simulink model "MMC_1ph_Grid_ArmLeaders_EnergyBalancing_v3_1A"  (R2024a)
settings: Solver=FixedStepDiscrete  StartTime=0.0  StopTime=1  FixedStep=Ts  RelTol=1e-3
PreLoadFcn:
  | VDC=800; N=8; C=2.2e-3; vo=100; W_nom=0.5*C*N*vo^2;
  | Larm=5e-3; Rarm=0.5; f=50;
  | Vg_rms=230; Vg_pk=Vg_rms*sqrt(2); Lg=2e-3; Rg=0.1;
  | Pstar=1500; Qstar=0;
  | fsw=1250; Ts=1e-5; Ts_ctrl=1e-4; Cf=10e-6; Rf=10;
InitFcn:
  | VDC=800; N=8; C=2.2e-3; vo=100; W_nom=0.5*C*N*vo^2;
  | Larm=5e-3; Rarm=0.5; f=50;
  | Vg_rms=230; Vg_pk=Vg_rms*sqrt(2); Lg=2e-3; Rg=0.1;
  | Pstar=1500; Qstar=0;
  | fsw=1250; Ts=1e-5; Ts_ctrl=1e-4; Cf=10e-6; Rf=10;
libraries: spsHalfBridgeMMCLib x16, spsSeriesRLCBranchLib x4, spsCurrentMeasurementLib x3, spsGroundLib x2, spsDCVoltageSourceLib x2, spsACVoltageSourceLib x1, spspowerguiLib x1, spsVoltageMeasurementLib x1
(part 2 of 2)

== matlab function MMC_1ph_Grid_ArmLeaders_EnergyBalancing_v3_1A/SM_l7/Local Ctrl ==
  data: sm_id input; S_top output; m_arm input; i_arm input; Vc_i input; Vc_prev input; Vc_next input; t input; S_bot output
function [S_top, S_bot] = hb_sm_local_ctrl(sm_id, m_arm, i_arm, Vc_i, Vc_prev, Vc_next, t)
%#codegen
% ============ SUBMODULE LAYER : local voltage balancing + PSC-PWM ============
% Fully local: own capacitor voltage, the two ring neighbours, the arm modulation
% index, the arm current (sign only) and the time base.  No sorting and no access
% to the full Vc vector.  Executes at Ts (10 us).

N      = 8;         % SMs per arm  -> carrier phase shift (sm_id-1)/N
fsw    = 1250;      % carrier frequency per SM -> N*fsw = 10 kHz effective per arm
k_v    = 0.2;       % balancing gain (1/V)
dead   = 0.1;       % V, dead-band against chattering
Iscale = 1.0;       % A, smooth sign of the arm current

%% 1. neighbour-average consensus correction
err  = 0.5*(Vc_prev + Vc_next) - Vc_i;
if abs(err) < dead, err = 0; end
dirn = tanh(i_arm/Iscale);    % > 0 : inserting charges C  (both arms: i measured top -> bottom)
dm   = k_v*err*dirn;
m_i  = min(max(m_arm + dm, 0), 1);

%% 2. phase-shifted triangular carrier (0 -> 1 -> 0)
tau = mod(t*fsw + (sm_id - 1)/N, 1);
car = 1 - abs(2*tau - 1);

%% 3. half-bridge gating
if m_i >= car
    S_top = 1; S_bot = 0;     % insert  (+Vc)
else
    S_top = 0; S_bot = 1;     % bypass  (0 V)
end
end

== matlab function MMC_1ph_Grid_ArmLeaders_EnergyBalancing_v3_1A/SM_u8/Neighbors ==
  data: Vc_arm input; Vc_i output; i input; Vc_prev output; Vc_next output
function [Vc_i, Vc_prev, Vc_next] = get_neighbors(Vc_arm, i)
%#codegen
% Models the neighbour-to-neighbour link of the ring: returns the own capacitor
% voltage and the voltages of the previous / next (circular) neighbours.
% Only these three scalars reach the local controller.
N = length(Vc_arm);
k = min(max(round(i), 1), N);
Vc_i = Vc_arm(k);
if k == 1
    Vc_prev = Vc_arm(N);      % circular: SM1's previous neighbour is SMN
    Vc_next = Vc_arm(2);
elseif k == N
    Vc_prev = Vc_arm(N-1);
    Vc_next = Vc_arm(1);      % circular: SMN's next neighbour is SM1
else
    Vc_prev = Vc_arm(k-1);
    Vc_next = Vc_arm(k+1);
end
end

== matlab function MMC_1ph_Grid_ArmLeaders_EnergyBalancing_v3_1A/SM_u8/Local Ctrl ==
  data: sm_id input; S_top output; m_arm input; i_arm input; Vc_i input; Vc_prev input; Vc_next input; t input; S_bot output
function [S_top, S_bot] = hb_sm_local_ctrl(sm_id, m_arm, i_arm, Vc_i, Vc_prev, Vc_next, t)
%#codegen
% ============ SUBMODULE LAYER : local voltage balancing + PSC-PWM ============
% Fully local: own capacitor voltage, the two ring neighbours, the arm modulation
% index, the arm current (sign only) and the time base.  No sorting and no access
% to the full Vc vector.  Executes at Ts (10 us).

N      = 8;         % SMs per arm  -> carrier phase shift (sm_id-1)/N
fsw    = 1250;      % carrier frequency per SM -> N*fsw = 10 kHz effective per arm
k_v    = 0.2;       % balancing gain (1/V)
dead   = 0.1;       % V, dead-band against chattering
Iscale = 1.0;       % A, smooth sign of the arm current

%% 1. neighbour-average consensus correction
err  = 0.5*(Vc_prev + Vc_next) - Vc_i;
if abs(err) < dead, err = 0; end
dirn = tanh(i_arm/Iscale);    % > 0 : inserting charges C  (both arms: i measured top -> bottom)
dm   = k_v*err*dirn;
m_i  = min(max(m_arm + dm, 0), 1);

%% 2. phase-shifted triangular carrier (0 -> 1 -> 0)
tau = mod(t*fsw + (sm_id - 1)/N, 1);
car = 1 - abs(2*tau - 1);

%% 3. half-bridge gating
if m_i >= car
    S_top = 1; S_bot = 0;     % insert  (+Vc)
else
    S_top = 0; S_bot = 1;     % bypass  (0 V)
end
end

== matlab function MMC_1ph_Grid_ArmLeaders_EnergyBalancing_v3_1A/SM_l8/Neighbors ==
  data: Vc_arm input; Vc_i output; i input; Vc_prev output; Vc_next output
function [Vc_i, Vc_prev, Vc_next] = get_neighbors(Vc_arm, i)
%#codegen
% Models the neighbour-to-neighbour link of the ring: returns the own capacitor
% voltage and the voltages of the previous / next (circular) neighbours.
% Only these three scalars reach the local controller.
N = length(Vc_arm);
k = min(max(round(i), 1), N);
Vc_i = Vc_arm(k);
if k == 1
    Vc_prev = Vc_arm(N);      % circular: SM1's previous neighbour is SMN
    Vc_next = Vc_arm(2);
elseif k == N
    Vc_prev = Vc_arm(N-1);
    Vc_next = Vc_arm(1);      % circular: SMN's next neighbour is SM1
else
    Vc_prev = Vc_arm(k-1);
    Vc_next = Vc_arm(k+1);
end
end

== matlab function MMC_1ph_Grid_ArmLeaders_EnergyBalancing_v3_1A/SM_l8/Local Ctrl ==
  data: sm_id input; S_top output; m_arm input; i_arm input; Vc_i input; Vc_prev input; Vc_next input; t input; S_bot output
function [S_top, S_bot] = hb_sm_local_ctrl(sm_id, m_arm, i_arm, Vc_i, Vc_prev, Vc_next, t)
%#codegen
% ============ SUBMODULE LAYER : local voltage balancing + PSC-PWM ============
% Fully local: own capacitor voltage, the two ring neighbours, the arm modulation
% index, the arm current (sign only) and the time base.  No sorting and no access
% to the full Vc vector.  Executes at Ts (10 us).

N      = 8;         % SMs per arm  -> carrier phase shift (sm_id-1)/N
fsw    = 1250;      % carrier frequency per SM -> N*fsw = 10 kHz effective per arm
k_v    = 0.2;       % balancing gain (1/V)
dead   = 0.1;       % V, dead-band against chattering
Iscale = 1.0;       % A, smooth sign of the arm current

%% 1. neighbour-average consensus correction
err  = 0.5*(Vc_prev + Vc_next) - Vc_i;
if abs(err) < dead, err = 0; end
dirn = tanh(i_arm/Iscale);    % > 0 : inserting charges C  (both arms: i measured top -> bottom)
dm   = k_v*err*dirn;
m_i  = min(max(m_arm + dm, 0), 1);

%% 2. phase-shifted triangular carrier (0 -> 1 -> 0)
tau = mod(t*fsw + (sm_id - 1)/N, 1);
car = 1 - abs(2*tau - 1);

%% 3. half-bridge gating
if m_i >= car
    S_top = 1; S_bot = 0;     % insert  (+Vc)
else
    S_top = 0; S_bot = 1;     % bypass  (0 V)
end
end

== matlab function MMC_1ph_Grid_ArmLeaders_EnergyBalancing_v3_1A/Meas Filter MA10 ==
  data: v_ac input; v_ac_f output; i_ac input; i_u input; i_l input; i_ac_f output; i_u_f output; i_l_f output
function [v_ac_f, i_ac_f, i_u_f, i_l_f] = meas_avg(v_ac, i_ac, i_u, i_l)
%#codegen
% Measurement conditioning for the 10 kHz control layer.
% 10-sample boxcar at Ts = 10 us  ->  exact nulls at 10 kHz (= N*fsw, the dominant
% PWM ripple of each arm) and at its multiples, so the Rate Transition blocks that
% follow do not alias the switching ripple into the control loops.
M = 10;
persistent buf idx
if isempty(buf), buf = zeros(M,4); idx = 1; end
buf(idx,:) = [v_ac, i_ac, i_u, i_l];
idx = idx + 1; if idx > M, idx = 1; end
y = sum(buf,1)/M;
v_ac_f = y(1);
i_ac_f = y(2);
i_u_f  = y(3);
i_l_f  = y(4);
end

== matlab function MMC_1ph_Grid_ArmLeaders_EnergyBalancing_v3_1A/Arm Leader UPPER/Outer Loop ==
  data: v_ac input; i_ac_ref output; i_ac input; Pstar input; Qstar input; t input; theta output; V_amp output; P_meas output; Q_meas output
function [i_ac_ref, theta, V_amp, P_meas, Q_meas] = mmc_outer_ctrl(v_ac, i_ac, Pstar, Qstar, t)
%#codegen
% ================= OUTER LOOP - GRID-CONNECTED P/Q CONTROL (one instance per arm) =================
% Executes at Ts_ctrl (Rate Transition blocks on every input pin the rate).
% Both arm leaders run this same deterministic code on the same measurements, so
% they produce an identical i_ac_ref without exchanging anything.
%
%   SOGI on v_ac and i_ac -> orthogonal (alpha, beta) components
%   SOGI-PLL (normalised)  -> theta locked to the PCC voltage (v_alpha = V_amp*cos(theta))
%   P = 0.5*(va*ia + vb*ib) ,  Q = 0.5*(va*ib - vb*ia)   [Q > 0 : current LEADS voltage, capacitive]
%   i_ac_ref = Ip*cos(theta) - Iq*sin(theta)
%
%   USE_PLL = false falls back to an internal 50 Hz oscillator (standalone resistive load).

Ts      = 1e-4;              % execution period (s) == Ts_ctrl in the workspace
f0      = 50;  w0 = 2*pi*f0;
USE_PLL = true;              % true : grid-connected (PLL on v_ac)   false : internal oscillator
NMA     = 200;               % 20 ms moving average on P and Q (nulls 50/100 Hz residuals)
T_START = 0.15;              % s, references held at zero until the PLL has locked
PQ_RAMP = 10000;             % W/s (var/s), reference ramp after T_START (soft start)

% --- SOGI and PLL
k_sogi  = 1.41;              % SOGI gain -> bandwidth ~ k*f0/2 = 35 Hz
Kp_pll  = 50;  Ki_pll = 1000;   % on vq/V_amp (p.u.) -> wn = 32 rad/s (5 Hz), zeta = 0.79
dw_max  = 2*pi*5;            % rad/s, PLL integrator limit (+-5 Hz)

% --- P and Q loops (plant: P = 0.5*V_amp*Ip, ~163 W/A at 325 V) -> f_bw ~ 5 Hz
Kp_pq   = 0.004;             % A/W   (loop gain 0.65 with the 10 ms MA delay)
Ki_pq   = 0.2;               % A/(W*s)
I_max   = 15;                % A, amplitude limit of each current component
P_max   = 3000;              % W
Q_max   = 2000;              % var
tau_v   = 0.01;              % s, LPF on the SOGI magnitude

persistent th pll_i vs1 vs2 is1 is2 Vf bufP bufQ idx xi_p xi_q
if isempty(th)
    th = 0; pll_i = 0; vs1 = 0; vs2 = 0; is1 = 0; is2 = 0; Vf = 300;
    bufP = zeros(NMA,1); bufQ = zeros(NMA,1); idx = 1;
    xi_p = 0; xi_q = 0;
end

%% 1. SOGI (voltage and current), symplectic Euler at 10 kHz (unity gain at w0; forward Euler gives +2.3 %)
vs1 = vs1 + Ts*(k_sogi*w0*(v_ac - vs1) - w0*vs2);
vs2 = vs2 + Ts*w0*vs1;
is1 = is1 + Ts*(k_sogi*w0*(i_ac - is1) - w0*is2);
is2 = is2 + Ts*w0*is1;
va = vs1; vb = vs2; ia = is1; ib = is2;

%% 2. amplitude and angle
Vn = max(sqrt(va^2 + vb^2), 20);
Vf = Vf + (Ts/(tau_v + Ts))*(Vn - Vf);
V_amp = Vf;
if USE_PLL
    vq    = (-sin(th)*va + cos(th)*vb)/Vn;            % normalised q-axis error (p.u.)
    pll_i = min(max(pll_i + Ki_pll*Ts*vq, -dw_max), dw_max);
    th    = mod(th + (w0 + Kp_pll*vq + pll_i)*Ts, 2*pi);
else
    th    = mod(w0*t, 2*pi);
end
theta = th;

%% 3. measured P and Q (instantaneous from alpha/beta, then 20 ms average)
bufP(idx) = 0.5*(va*ia + vb*ib);
bufQ(idx) = 0.5*(va*ib - vb*ia);
idx = idx + 1; if idx > NMA, idx = 1; end
P_meas = sum(bufP)/NMA;
Q_meas = sum(bufQ)/NMA;

%% 4. P and Q loops -> current components (feed-forward + PI, clamping anti-windup)
if t < T_START
    P_use = 0; Q_use = 0;                             % wait for PLL lock
else
    lim   = PQ_RAMP*(t - T_START);                    % ramped envelope
    P_use = min(max(min(max(Pstar, -P_max), P_max), -lim), lim);
    Q_use = min(max(min(max(Qstar, -Q_max), Q_max), -lim), lim);
end
Ip_ff = 2*P_use/V_amp;   Iq_ff = 2*Q_use/V_amp;
e_p = P_use - P_meas;    e_q = Q_use - Q_meas;
Ip_un = Ip_ff + Kp_pq*e_p + xi_p;
if abs(Ip_un) < I_max, xi_p = min(max(xi_p + Ki_pq*Ts*e_p, -I_max), I_max); end
Iq_un = Iq_ff + Kp_pq*e_q + xi_q;
if abs(Iq_un) < I_max, xi_q = min(max(xi_q + Ki_pq*Ts*e_q, -I_max), I_max); end
Ip = min(max(Ip_un, -I_max), I_max);
Iq = min(max(Iq_un, -I_max), I_max);

%% 5. AC current reference
i_ac_ref = Ip*cos(theta) - Iq*sin(theta);
end

== matlab function MMC_1ph_Grid_ArmLeaders_EnergyBalancing_v3_1A/SM_l1/Neighbors ==
  data: Vc_arm input; Vc_i output; i input; Vc_prev output; Vc_next output
function [Vc_i, Vc_prev, Vc_next] = get_neighbors(Vc_arm, i)
%#codegen
% Models the neighbour-to-neighbour link of the ring: returns the own capacitor
% voltage and the voltages of the previous / next (circular) neighbours.
% Only these three scalars reach the local controller.
N = length(Vc_arm);
k = min(max(round(i), 1), N);
Vc_i = Vc_arm(k);
if k == 1
    Vc_prev = Vc_arm(N);      % circular: SM1's previous neighbour is SMN
    Vc_next = Vc_arm(2);
elseif k == N
    Vc_prev = Vc_arm(N-1);
    Vc_next = Vc_arm(1);      % circular: SMN's next neighbour is SM1
else
    Vc_prev = Vc_arm(k-1);
    Vc_next = Vc_arm(k+1);
end
end

== matlab function MMC_1ph_Grid_ArmLeaders_EnergyBalancing_v3_1A/Arm Leader UPPER/Inner Loop and Energy Balancing ==
  data: i_ac_ref input; m_arm output; theta input; V_amp input; P_meas input; v_ac input; i_arm input; Vc_arm input; W_other input; IsUpper input; Vdc input; Vc_nom input; W_arm output; dbg output
function [m_arm, W_arm, dbg] = mmc_arm_ctrl(i_ac_ref, theta, V_amp, P_meas, v_ac, i_arm, Vc_arm, W_other, IsUpper, Vdc, Vc_nom)
%#codegen
% ========== INNER LOOP + INTER-ARM ENERGY BALANCING  (one instance per arm) ==========
% Executes at Ts_ctrl.  The only information this arm needs from the OTHER arm is
% one scalar: its raw stored energy W_other (received through a one-period unit
% delay that models the communication latency).  With s = +1 (upper) / -1 (lower)
% both leaders compute the SAME i_circ_ref, so no further coordination is needed.
%
%   m_arm : modulation index of this arm (0..1)      -> SM layer (local PSC-PWM)
%   W_arm : raw energy of this arm (J)               -> sent to the other arm
%   dbg   : [i_ref; i_circ_ref; v_arm_ref; W_own_f; W_other_f]
%   Vdc, Vc_nom : DC-link voltage and nominal SM voltage, read from the workspace (VDC, vo)
%                 through Constant blocks.  N*Vc_nom may exceed Vdc (stack margin for |v_ac| -> Vdc/2).

Ts     = 1e-4;
C      = 2.2e-3;
N      = numel(Vc_arm);
w0     = 2*pi*50;
NMA    = 200;                 % 20 ms moving average on the energies (nulls 50/100 Hz)

% --- arm current loop: PI + resonant terms at 50 Hz and 100 Hz (plant L = 5 mH, R = 0.5 ohm) -> f_bw ~ 380 Hz
Kp_i = 12;    Ki_i = 1200;    Kr_i = 300;   xi_i_max = 300;   xr_max = 200;   v_pi_max = 400;
% --- CCSC: resonant term at 2*w0 removes the 100 Hz circulating current from THIS arm's current.
%     i_ref carries no 2w0 component, so any 2w0 content of i_arm is error -> driven to zero locally,
%     without knowing the other arm's current (single-phase equivalent of the dq -2w CCSC).
USE_CCSC = true;   Kr_2 = 300;   xr2_max = 150;
% --- total-energy loop  (dW_sum/dt = Vdc*i_dc - P_ac)          -> f_bw ~ 4 Hz
Kp_s = 0.03;  Ki_s = 0.3;     xi_s_max = 3;     i_dc_max  = 5;
% --- differential-energy loop (dW_dif/dt = -V_amp*I_dif)       -> wn ~ 12 rad/s, critically damped
Kp_d = 25;    Ki_d = 150;     xi_d_max = 300;   I_dif_max = 3;

persistent xi_i xr1 xr2 xc1 xc2 xi_s xi_d bufO bufX idx
if isempty(xi_i)
    xi_i = 0; xr1 = 0; xr2 = 0; xc1 = 0; xc2 = 0; xi_s = 0; xi_d = 0;
    W0   = 0.5*C*N*Vc_nom^2;
    bufO = W0*ones(NMA,1); bufX = W0*ones(NMA,1); idx = 1;
end
if IsUpper > 0.5, s = 1; else, s = -1; end

%% 1. own arm energy (raw) -> exported to the other arm
W_arm = 0.5*C*sum(Vc_arm.^2);
W_nom = 0.5*C*N*Vc_nom^2;

%% 2. energy filtering (both arms use identical filters -> identical results)
bufO(idx) = W_arm;
bufX(idx) = W_other;
idx = idx + 1; if idx > NMA, idx = 1; end
Wo = sum(bufO)/NMA;           % own   (filtered)
Wx = sum(bufX)/NMA;           % other (filtered)

%% 3. energy-balancing layer
% 3a. total energy -> DC circulating current (identical in both arms)
e_sum   = 2*W_nom - (Wo + Wx);
i_dc_un = P_meas/Vdc + Kp_s*e_sum + xi_s;                        % unsaturated
if abs(i_dc_un) < i_dc_max                                       % clamping anti-windup
    xi_s = min(max(xi_s + Ki_s*Ts*e_sum, -xi_s_max), xi_s_max);
end
i_dc_ref = min(max(i_dc_un, -i_dc_max), i_dc_max);

% 3b. differential energy (own - other) -> fundamental circulating current in phase
%     with v_ac.  s flips the sign so that both arms demand the SAME I_dif:
%     upper: +K*(Wu-Wl)   lower: -K*(Wl-Wu) = +K*(Wu-Wl)
e_dif    = Wo - Wx;
u_dif    = Kp_d*e_dif + xi_d;                                    % W
I_dif_un = s*u_dif/max(V_amp, 50);                               % A (unsaturated)
if abs(I_dif_un) < I_dif_max                                     % clamping anti-windup
    xi_d = min(max(xi_d + Ki_d*Ts*e_dif, -xi_d_max), xi_d_max);
end
I_dif = min(max(I_dif_un, -I_dif_max), I_dif_max);
i_circ_ref = i_dc_ref + I_dif*cos(theta);

%% 4. arm current reference and inner PI + R
%     i_u = +i_ac/2 + i_circ ,  i_l = -i_ac/2 + i_circ   (both measured top -> bottom)
i_ref = s*0.5*i_ac_ref + i_circ_ref;
err_i = i_ref - i_arm;
xi_i  = min(max(xi_i + Ki_i*Ts*err_i, -xi_i_max), xi_i_max);
% resonant integrator at w0 (symplectic Euler: |lambda| = 1, no drift)
xr1   = xr1 + Ts*(Kr_i*err_i - w0*xr2);
xr2   = xr2 + Ts*w0*xr1;
xr1   = min(max(xr1, -xr_max), xr_max);
% resonant integrator at 2*w0 (CCSC)
if USE_CCSC
    xc1 = xc1 + Ts*(Kr_2*err_i - 2*w0*xc2);
    xc2 = xc2 + Ts*2*w0*xc1;
    xc1 = min(max(xc1, -xr2_max), xr2_max);
else
    xc1 = 0; xc2 = 0;
end
v_pi  = min(max(Kp_i*err_i + xi_i + xr1 + xc1, -v_pi_max), v_pi_max);

%% 5. arm voltage reference -> modulation index
%     upper: v_u = Vdc/2 - v_ac - v_pi      lower: v_l = Vdc/2 + v_ac - v_pi
v_arm_ref = Vdc/2 - s*v_ac - v_pi;
V_stack   = max(sum(Vc_arm), 0.5*N*Vc_nom);        % measured stack voltage
m_arm     = min(max(v_arm_ref/V_stack, 0), 1);

dbg = [i_ref; i_circ_ref; v_arm_ref; Wo; Wx];
end

== matlab function MMC_1ph_Grid_ArmLeaders_EnergyBalancing_v3_1A/Arm Leader LOWER/Outer Loop ==
  data: v_ac input; i_ac_ref output; i_ac input; Pstar input; Qstar input; t input; theta output; V_amp output; P_meas output; Q_meas output
function [i_ac_ref, theta, V_amp, P_meas, Q_meas] = mmc_outer_ctrl(v_ac, i_ac, Pstar, Qstar, t)
%#codegen
% ================= OUTER LOOP - GRID-CONNECTED P/Q CONTROL (one instance per arm) =================
% Executes at Ts_ctrl (Rate Transition blocks on every input pin the rate).
% Both arm leaders run this same deterministic code on the same measurements, so
% they produce an identical i_ac_ref without exchanging anything.
%
%   SOGI on v_ac and i_ac -> orthogonal (alpha, beta) components
%   SOGI-PLL (normalised)  -> theta locked to the PCC voltage (v_alpha = V_amp*cos(theta))
%   P = 0.5*(va*ia + vb*ib) ,  Q = 0.5*(va*ib - vb*ia)   [Q > 0 : current LEADS voltage, capacitive]
%   i_ac_ref = Ip*cos(theta) - Iq*sin(theta)
%
%   USE_PLL = false falls back to an internal 50 Hz oscillator (standalone resistive load).

Ts      = 1e-4;              % execution period (s) == Ts_ctrl in the workspace
f0      = 50;  w0 = 2*pi*f0;
USE_PLL = true;              % true : grid-connected (PLL on v_ac)   false : internal oscillator
NMA     = 200;               % 20 ms moving average on P and Q (nulls 50/100 Hz residuals)
T_START = 0.15;              % s, references held at zero until the PLL has locked
PQ_RAMP = 10000;             % W/s (var/s), reference ramp after T_START (soft start)

% --- SOGI and PLL
k_sogi  = 1.41;              % SOGI gain -> bandwidth ~ k*f0/2 = 35 Hz
Kp_pll  = 50;  Ki_pll = 1000;   % on vq/V_amp (p.u.) -> wn = 32 rad/s (5 Hz), zeta = 0.79
dw_max  = 2*pi*5;            % rad/s, PLL integrator limit (+-5 Hz)

% --- P and Q loops (plant: P = 0.5*V_amp*Ip, ~163 W/A at 325 V) -> f_bw ~ 5 Hz
Kp_pq   = 0.004;             % A/W   (loop gain 0.65 with the 10 ms MA delay)
Ki_pq   = 0.2;               % A/(W*s)
I_max   = 15;                % A, amplitude limit of each current component
P_max   = 3000;              % W
Q_max   = 2000;              % var
tau_v   = 0.01;              % s, LPF on the SOGI magnitude

persistent th pll_i vs1 vs2 is1 is2 Vf bufP bufQ idx xi_p xi_q
if isempty(th)
    th = 0; pll_i = 0; vs1 = 0; vs2 = 0; is1 = 0; is2 = 0; Vf = 300;
    bufP = zeros(NMA,1); bufQ = zeros(NMA,1); idx = 1;
    xi_p = 0; xi_q = 0;
end

%% 1. SOGI (voltage and current), symplectic Euler at 10 kHz (unity gain at w0; forward Euler gives +2.3 %)
vs1 = vs1 + Ts*(k_sogi*w0*(v_ac - vs1) - w0*vs2);
vs2 = vs2 + Ts*w0*vs1;
is1 = is1 + Ts*(k_sogi*w0*(i_ac - is1) - w0*is2);
is2 = is2 + Ts*w0*is1;
va = vs1; vb = vs2; ia = is1; ib = is2;

%% 2. amplitude and angle
Vn = max(sqrt(va^2 + vb^2), 20);
Vf = Vf + (Ts/(tau_v + Ts))*(Vn - Vf);
V_amp = Vf;
if USE_PLL
    vq    = (-sin(th)*va + cos(th)*vb)/Vn;            % normalised q-axis error (p.u.)
    pll_i = min(max(pll_i + Ki_pll*Ts*vq, -dw_max), dw_max);
    th    = mod(th + (w0 + Kp_pll*vq + pll_i)*Ts, 2*pi);
else
    th    = mod(w0*t, 2*pi);
end
theta = th;

%% 3. measured P and Q (instantaneous from alpha/beta, then 20 ms average)
bufP(idx) = 0.5*(va*ia + vb*ib);
bufQ(idx) = 0.5*(va*ib - vb*ia);
idx = idx + 1; if idx > NMA, idx = 1; end
P_meas = sum(bufP)/NMA;
Q_meas = sum(bufQ)/NMA;

%% 4. P and Q loops -> current components (feed-forward + PI, clamping anti-windup)
if t < T_START
    P_use = 0; Q_use = 0;                             % wait for PLL lock
else
    lim   = PQ_RAMP*(t - T_START);                    % ramped envelope
    P_use = min(max(min(max(Pstar, -P_max), P_max), -lim), lim);
    Q_use = min(max(min(max(Qstar, -Q_max), Q_max), -lim), lim);
end
Ip_ff = 2*P_use/V_amp;   Iq_ff = 2*Q_use/V_amp;
e_p = P_use - P_meas;    e_q = Q_use - Q_meas;
Ip_un = Ip_ff + Kp_pq*e_p + xi_p;
if abs(Ip_un) < I_max, xi_p = min(max(xi_p + Ki_pq*Ts*e_p, -I_max), I_max); end
Iq_un = Iq_ff + Kp_pq*e_q + xi_q;
if abs(Iq_un) < I_max, xi_q = min(max(xi_q + Ki_pq*Ts*e_q, -I_max), I_max); end
Ip = min(max(Ip_un, -I_max), I_max);
Iq = min(max(Iq_un, -I_max), I_max);

%% 5. AC current reference
i_ac_ref = Ip*cos(theta) - Iq*sin(theta);
end

== matlab function MMC_1ph_Grid_ArmLeaders_EnergyBalancing_v3_1A/Arm Leader LOWER/Inner Loop and Energy Balancing ==
  data: i_ac_ref input; m_arm output; theta input; V_amp input; P_meas input; v_ac input; i_arm input; Vc_arm input; W_other input; IsUpper input; Vdc input; Vc_nom input; W_arm output; dbg output
function [m_arm, W_arm, dbg] = mmc_arm_ctrl(i_ac_ref, theta, V_amp, P_meas, v_ac, i_arm, Vc_arm, W_other, IsUpper, Vdc, Vc_nom)
%#codegen
% ========== INNER LOOP + INTER-ARM ENERGY BALANCING  (one instance per arm) ==========
% Executes at Ts_ctrl.  The only information this arm needs from the OTHER arm is
% one scalar: its raw stored energy W_other (received through a one-period unit
% delay that models the communication latency).  With s = +1 (upper) / -1 (lower)
% both leaders compute the SAME i_circ_ref, so no further coordination is needed.
%
%   m_arm : modulation index of this arm (0..1)      -> SM layer (local PSC-PWM)
%   W_arm : raw energy of this arm (J)               -> sent to the other arm
%   dbg   : [i_ref; i_circ_ref; v_arm_ref; W_own_f; W_other_f]
%   Vdc, Vc_nom : DC-link voltage and nominal SM voltage, read from the workspace (VDC, vo)
%                 through Constant blocks.  N*Vc_nom may exceed Vdc (stack margin for |v_ac| -> Vdc/2).

Ts     = 1e-4;
C      = 2.2e-3;
N      = numel(Vc_arm);
w0     = 2*pi*50;
NMA    = 200;                 % 20 ms moving average on the energies (nulls 50/100 Hz)

% --- arm current loop: PI + resonant terms at 50 Hz and 100 Hz (plant L = 5 mH, R = 0.5 ohm) -> f_bw ~ 380 Hz
Kp_i = 12;    Ki_i = 1200;    Kr_i = 300;   xi_i_max = 300;   xr_max = 200;   v_pi_max = 400;
% --- CCSC: resonant term at 2*w0 removes the 100 Hz circulating current from THIS arm's current.
%     i_ref carries no 2w0 component, so any 2w0 content of i_arm is error -> driven to zero locally,
%     without knowing the other arm's current (single-phase equivalent of the dq -2w CCSC).
USE_CCSC = true;   Kr_2 = 300;   xr2_max = 150;
% --- total-energy loop  (dW_sum/dt = Vdc*i_dc - P_ac)          -> f_bw ~ 4 Hz
Kp_s = 0.03;  Ki_s = 0.3;     xi_s_max = 3;     i_dc_max  = 5;
% --- differential-energy loop (dW_dif/dt = -V_amp*I_dif)       -> wn ~ 12 rad/s, critically damped
Kp_d = 25;    Ki_d = 150;     xi_d_max = 300;   I_dif_max = 3;

persistent xi_i xr1 xr2 xc1 xc2 xi_s xi_d bufO bufX idx
if isempty(xi_i)
    xi_i = 0; xr1 = 0; xr2 = 0; xc1 = 0; xc2 = 0; xi_s = 0; xi_d = 0;
    W0   = 0.5*C*N*Vc_nom^2;
    bufO = W0*ones(NMA,1); bufX = W0*ones(NMA,1); idx = 1;
end
if IsUpper > 0.5, s = 1; else, s = -1; end

%% 1. own arm energy (raw) -> exported to the other arm
W_arm = 0.5*C*sum(Vc_arm.^2);
W_nom = 0.5*C*N*Vc_nom^2;

%% 2. energy filtering (both arms use identical filters -> identical results)
bufO(idx) = W_arm;
bufX(idx) = W_other;
idx = idx + 1; if idx > NMA, idx = 1; end
Wo = sum(bufO)/NMA;           % own   (filtered)
Wx = sum(bufX)/NMA;           % other (filtered)

%% 3. energy-balancing layer
% 3a. total energy -> DC circulating current (identical in both arms)
e_sum   = 2*W_nom - (Wo + Wx);
i_dc_un = P_meas/Vdc + Kp_s*e_sum + xi_s;                        % unsaturated
if abs(i_dc_un) < i_dc_max                                       % clamping anti-windup
    xi_s = min(max(xi_s + Ki_s*Ts*e_sum, -xi_s_max), xi_s_max);
end
i_dc_ref = min(max(i_dc_un, -i_dc_max), i_dc_max);

% 3b. differential energy (own - other) -> fundamental circulating current in phase
%     with v_ac.  s flips the sign so that both arms demand the SAME I_dif:
%     upper: +K*(Wu-Wl)   lower: -K*(Wl-Wu) = +K*(Wu-Wl)
e_dif    = Wo - Wx;
u_dif    = Kp_d*e_dif + xi_d;                                    % W
I_dif_un = s*u_dif/max(V_amp, 50);                               % A (unsaturated)
if abs(I_dif_un) < I_dif_max                                     % clamping anti-windup
    xi_d = min(max(xi_d + Ki_d*Ts*e_dif, -xi_d_max), xi_d_max);
end
I_dif = min(max(I_dif_un, -I_dif_max), I_dif_max);
i_circ_ref = i_dc_ref + I_dif*cos(theta);

%% 4. arm current reference and inner PI + R
%     i_u = +i_ac/2 + i_circ ,  i_l = -i_ac/2 + i_circ   (both measured top -> bottom)
i_ref = s*0.5*i_ac_ref + i_circ_ref;
err_i = i_ref - i_arm;
xi_i  = min(max(xi_i + Ki_i*Ts*err_i, -xi_i_max), xi_i_max);
% resonant integrator at w0 (symplectic Euler: |lambda| = 1, no drift)
xr1   = xr1 + Ts*(Kr_i*err_i - w0*xr2);
xr2   = xr2 + Ts*w0*xr1;
xr1   = min(max(xr1, -xr_max), xr_max);
% resonant integrator at 2*w0 (CCSC)
if USE_CCSC
    xc1 = xc1 + Ts*(Kr_2*err_i - 2*w0*xc2);
    xc2 = xc2 + Ts*2*w0*xc1;
    xc1 = min(max(xc1, -xr2_max), xr2_max);
else
    xc1 = 0; xc2 = 0;
end
v_pi  = min(max(Kp_i*err_i + xi_i + xr1 + xc1, -v_pi_max), v_pi_max);

%% 5. arm voltage reference -> modulation index
%     upper: v_u = Vdc/2 - v_ac - v_pi      lower: v_l = Vdc/2 + v_ac - v_pi
v_arm_ref = Vdc/2 - s*v_ac - v_pi;
V_stack   = max(sum(Vc_arm), 0.5*N*Vc_nom);        % measured stack voltage
m_arm     = min(max(v_arm_ref/V_stack, 0), 1);

dbg = [i_ref; i_circ_ref; v_arm_ref; Wo; Wx];
end

== matlab function MMC_1ph_Grid_ArmLeaders_EnergyBalancing_v3_1A/SM_l1/Local Ctrl ==
  data: sm_id input; S_top output; m_arm input; i_arm input; Vc_i input; Vc_prev input; Vc_next input; t input; S_bot output
function [S_top, S_bot] = hb_sm_local_ctrl(sm_id, m_arm, i_arm, Vc_i, Vc_prev, Vc_next, t)
%#codegen
% ============ SUBMODULE LAYER : local voltage balancing + PSC-PWM ============
% Fully local: own capacitor voltage, the two ring neighbours, the arm modulation
% index, the arm current (sign only) and the time base.  No sorting and no access
% to the full Vc vector.  Executes at Ts (10 us).

N      = 8;         % SMs per arm  -> carrier phase shift (sm_id-1)/N
fsw    = 1250;      % carrier frequency per SM -> N*fsw = 10 kHz effective per arm
k_v    = 0.2;       % balancing gain (1/V)
dead   = 0.1;       % V, dead-band against chattering
Iscale = 1.0;       % A, smooth sign of the arm current

%% 1. neighbour-average consensus correction
err  = 0.5*(Vc_prev + Vc_next) - Vc_i;
if abs(err) < dead, err = 0; end
dirn = tanh(i_arm/Iscale);    % > 0 : inserting charges C  (both arms: i measured top -> bottom)
dm   = k_v*err*dirn;
m_i  = min(max(m_arm + dm, 0), 1);

%% 2. phase-shifted triangular carrier (0 -> 1 -> 0)
tau = mod(t*fsw + (sm_id - 1)/N, 1);
car = 1 - abs(2*tau - 1);

%% 3. half-bridge gating
if m_i >= car
    S_top = 1; S_bot = 0;     % insert  (+Vc)
else
    S_top = 0; S_bot = 1;     % bypass  (0 V)
end
end

== matlab function MMC_1ph_Grid_ArmLeaders_EnergyBalancing_v3_1A/SM_u2/Neighbors ==
  data: Vc_arm input; Vc_i output; i input; Vc_prev output; Vc_next output
function [Vc_i, Vc_prev, Vc_next] = get_neighbors(Vc_arm, i)
%#codegen
% Models the neighbour-to-neighbour link of the ring: returns the own capacitor
% voltage and the voltages of the previous / next (circular) neighbours.
% Only these three scalars reach the local controller.
N = length(Vc_arm);
k = min(max(round(i), 1), N);
Vc_i = Vc_arm(k);
if k == 1
    Vc_prev = Vc_arm(N);      % circular: SM1's previous neighbour is SMN
    Vc_next = Vc_arm(2);
elseif k == N
    Vc_prev = Vc_arm(N-1);
    Vc_next = Vc_arm(1);      % circular: SMN's next neighbour is SM1
else
    Vc_prev = Vc_arm(k-1);
    Vc_next = Vc_arm(k+1);
end
end

== matlab function MMC_1ph_Grid_ArmLeaders_EnergyBalancing_v3_1A/SM_u2/Local Ctrl ==
  data: sm_id input; S_top output; m_arm input; i_arm input; Vc_i input; Vc_prev input; Vc_next input; t input; S_bot output
function [S_top, S_bot] = hb_sm_local_ctrl(sm_id, m_arm, i_arm, Vc_i, Vc_prev, Vc_next, t)
%#codegen
% ============ SUBMODULE LAYER : local voltage balancing + PSC-PWM ============
% Fully local: own capacitor voltage, the two ring neighbours, the arm modulation
% index, the arm current (sign only) and the time base.  No sorting and no access
% to the full Vc vector.  Executes at Ts (10 us).

N      = 8;         % SMs per arm  -> carrier phase shift (sm_id-1)/N
fsw    = 1250;      % carrier frequency per SM -> N*fsw = 10 kHz effective per arm
k_v    = 0.2;       % balancing gain (1/V)
dead   = 0.1;       % V, dead-band against chattering
Iscale = 1.0;       % A, smooth sign of the arm current

%% 1. neighbour-average consensus correction
err  = 0.5*(Vc_prev + Vc_next) - Vc_i;
if abs(err) < dead, err = 0; end
dirn = tanh(i_arm/Iscale);    % > 0 : inserting charges C  (both arms: i measured top -> bottom)
dm   = k_v*err*dirn;
m_i  = min(max(m_arm + dm, 0), 1);

%% 2. phase-shifted triangular carrier (0 -> 1 -> 0)
tau = mod(t*fsw + (sm_id - 1)/N, 1);
car = 1 - abs(2*tau - 1);

%% 3. half-bridge gating
if m_i >= car
    S_top = 1; S_bot = 0;     % insert  (+Vc)
else
    S_top = 0; S_bot = 1;     % bypass  (0 V)
end
end

== matlab function MMC_1ph_Grid_ArmLeaders_EnergyBalancing_v3_1A/SM_l2/Neighbors ==
  data: Vc_arm input; Vc_i output; i input; Vc_prev output; Vc_next output
function [Vc_i, Vc_prev, Vc_next] = get_neighbors(Vc_arm, i)
%#codegen
% Models the neighbour-to-neighbour link of the ring: returns the own capacitor
% voltage and the voltages of the previous / next (circular) neighbours.
% Only these three scalars reach the local controller.
N = length(Vc_arm);
k = min(max(round(i), 1), N);
Vc_i = Vc_arm(k);
if k == 1
    Vc_prev = Vc_arm(N);      % circular: SM1's previous neighbour is SMN
    Vc_next = Vc_arm(2);
elseif k == N
    Vc_prev = Vc_arm(N-1);
    Vc_next = Vc_arm(1);      % circular: SMN's next neighbour is SM1
else
    Vc_prev = Vc_arm(k-1);
    Vc_next = Vc_arm(k+1);
end
end
